simulink model "Range_ext_TCST_NoSDKF"  (R2024b)
settings: Solver=ode1  StartTime=0.0  StopTime=110000  FixedStep=5  RelTol=1e-3  EnableMultiTasking=on
values from neighbouring files (symbols this model uses):
  delta = 5    [Range_Max_2.m]    (also in Sim_Run.m; Sim_Run_Auto.m; Sim_Run_Auto_Static_SOC.m; Sim_Run_conflict_copy_danishs-macbook-air_2025_03_05.m)
  Stop_SOC = 0.1    [Sim_Run.m]    (also in Sim_Run_Auto.m; Sim_Run_Auto_Static_SOC.m; Sim_Run_conflict_copy_danishs-macbook-air_2025_03_05.m; comparison_test_weights.m)
  weights = [0.0;0.35;0.96;w_PL]    [Sim_Run.m]    (also in Sim_Run_Auto.m = [w1; w2; w3; w_PL]; Sim_Run_Auto_Static_SOC.m = [w1; w2; w3; w_PL]; Sim_Run_conflict_copy_danishs-macbook-air_2025_03_05.m = [1.0;0;0;w_PL]; comparison_test_weights.m = [w1; w2; w3; w_PL])
  x_0 = [H;M;L]    [Sim_Run.m]    (also in Sim_Run_Auto.m = [H; M; L]; Sim_Run_Auto_Static_SOC.m = [H; M; L]; Sim_Run_conflict_copy_danishs-macbook-air_2025_03_05.m; comparison_test_weights.m = [H; M; L])
settings Model: Creator=jgillis  LastModifiedBy=danish
settings SolverCC: ZeroCrossControl=DisableAll  AlgebraicLoopSolver=TrustRegion
settings DataIOCC: SaveFormat=Array  ReturnWorkspaceOutputs=off
settings OptimizationCC: LifeSpan=inf
settings DebuggingCC: UnconnectedInputMsg=warning  UnconnectedOutputMsg=warning  UnconnectedLineMsg=warning  SFUnexpectedBacktrackingDiag=warning  SFNoUnconditionalDefaultTransitionDiag=warning  ArithmeticOperatorsInVariantConditions=warning
settings HardwareCC: ProdBitPerPointer=32  ProdBitPerSizeT=32  ProdBitPerPtrDiffT=32  ProdLargestAtomicFloat=None  ProdIntDivRoundTo=Undefined  ProdEndianess=Unspecified  ProdWordSize=32  ProdHWDeviceType=32-bit Generic
settings ModelReferenceCC: EnableRefExpFcnMdlSchedulingChecks=on  PropagateSignalLabelsOutOfModel=off
settings SFSimCC: SimUseLocalCustomCode=off  CustomCodeUndefinedFunction=UseInterfaceOnly
settings RTWCC: RTWUseLocalCustomCode=off  GPUComputeCapability=3.5
settings CodeAppCC: StateflowObjectComments=on
settings GRTTargetCC: TargetLangStandard=C89/C90 (ANSI)
settings ConfigComp: CovMetricSettings=dw  CovSaveCumulativeToWorkspaceVar=on  CovSaveSingleToWorkspaceVar=on  CovExternalEMLEnable=off  CovSFcnEnable=off

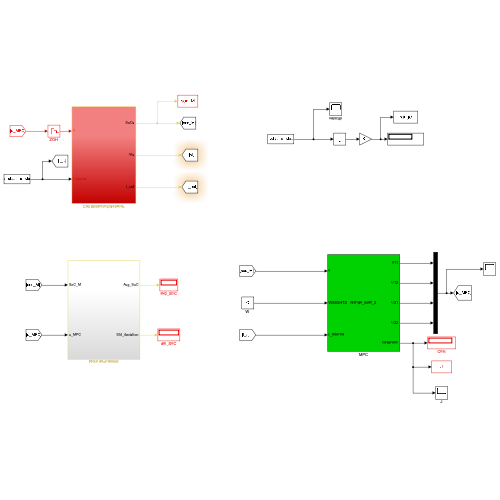
[thumbnail: Simulink's stored preview of the top-level diagram]
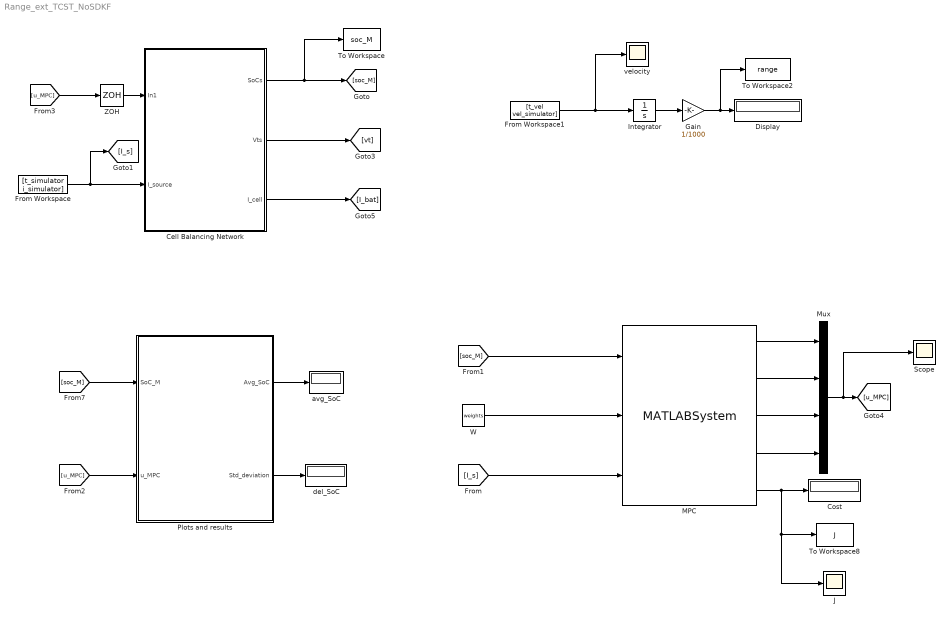
== system Range_ext_TCST_NoSDKF ==
  Cell Balancing Network : Subsystem
  Cost : Display
  Display : Display
  From Workspace : FromWorkspace  VariableName=[t_simulator i_simulator]  SampleTime=-1
  From Workspace1 : FromWorkspace  VariableName=[t_vel vel_simulator]  SampleTime=-1
  Gain : Gain  Gain=1/1000
  Integrator : Integrator
  J : Scope
  MPC : MATLABSystem  System=Range_Max_2  SimulateUsing=Interpreted execution
      mask Type: Range_Max_2
      mask Display:
      | disp('Range_Max_2');
      | port_label('input',1,'x');
      | port_label('input',2,'WEIGHTS');
      | port_label('input',3,'I_source');
      | port_label('output',1,'u11');
      | port_label('output',2,'u12');
      | port_label('output',3,'u21');
      | port_label('output',4,'u22');
      | port_label('output',5,'costFunc');
  Mux : Mux
  Plots and results : Subsystem
  Scope : Scope
  To Workspace : ToWorkspace  VariableName=soc_M  SampleTime=-1
      settings: Save2DSignal=2-D array (concatenate along first dimension)
  To Workspace2 : ToWorkspace  VariableName=range  SampleTime=-1
      settings: Save2DSignal=2-D array (concatenate along first dimension)
  To Workspace8 : ToWorkspace  VariableName=J  SampleTime=-1
      settings: Save2DSignal=2-D array (concatenate along first dimension)
  W : Constant  Value=weights
  ZOH : ZeroOrderHold  SampleTime=delta
  avg_SoC : Display
  del_SoC : Display
  velocity : Scope
  wires:
  Cell Balancing Network/2(Vts) -> [vt]
  Cell Balancing Network/1(SoCs) -> To Workspace/1, [soc_M]
  Cell Balancing Network/3(I_cell) -> [I_bat]
  [soc_M] -> MPC/1
  MPC/4 -> Mux/4
  MPC/3 -> Mux/3
  MPC/2 -> Mux/2
  MPC/1 -> Mux/1
  Mux/1 -> Scope/1, [u_MPC]
  MPC/5 -> To Workspace8/1, J/1, Cost/1
  [soc_M] -> Plots and results/1(SoC_M)
  Plots and results/1(Avg_SoC) -> avg_SoC/1
  Plots and results/2(Std_deviation) -> del_SoC/1
  ZOH/1 -> Cell Balancing Network/1(In1)
  [u_MPC] -> Plots and results/2(u_MPC)
  From Workspace1/1 -> velocity/1, Integrator/1
  Integrator/1 -> Gain/1
  Gain/1 -> To Workspace2/1, Display/1
  From Workspace/1 -> [I_s], Cell Balancing Network/2(I_source)
  [u_MPC] -> ZOH/1
  [I_s] -> MPC/3
  W/1 -> MPC/2

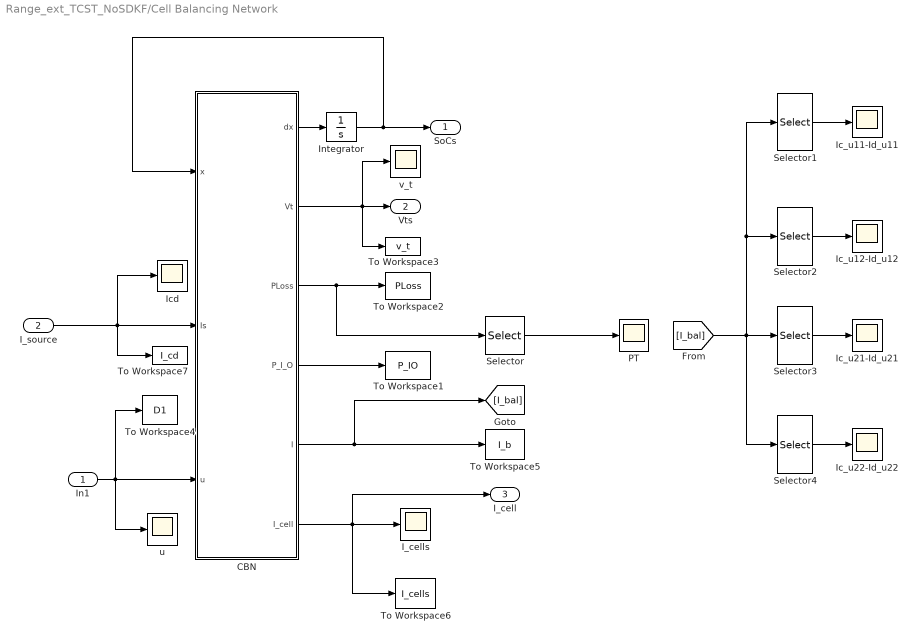
== system Range_ext_TCST_NoSDKF/Cell Balancing Network ==
  In1 : Inport
  I_source : Inport  Port=2
  CBN : MATLAB Function  TreatAsAtomicUnit=on
  I_cells : Scope
  Ic_u11-Id_u11 : Scope
  Ic_u12-Id_u12 : Scope
  Ic_u21-Id_u21 : Scope
  Ic_u22-Id_u22 : Scope
  Icd : Scope
  Integrator : Integrator  InitialCondition=x_0
  PT : Scope
  Selector : Selector  InputPortWidth=5  IndexOptions=Index vector (dialog)  Indices=1  OutputSizes=1
  Selector1 : Selector  InputPortWidth=8  IndexOptions=Index vector (dialog)  Indices=[1 2]  OutputSizes=1
  Selector2 : Selector  InputPortWidth=8  IndexOptions=Index vector (dialog)  Indices=[3 4]  OutputSizes=1
  Selector3 : Selector  InputPortWidth=8  IndexOptions=Index vector (dialog)  Indices=[5 6]  OutputSizes=1
  Selector4 : Selector  InputPortWidth=8  IndexOptions=Index vector (dialog)  Indices=[7 8]  OutputSizes=1
  To Workspace1 : ToWorkspace  VariableName=P_IO  SampleTime=-1
      settings: Save2DSignal=2-D array (concatenate along first dimension)
  To Workspace2 : ToWorkspace  VariableName=PLoss  SampleTime=-1
      settings: Save2DSignal=2-D array (concatenate along first dimension)
  To Workspace3 : ToWorkspace  VariableName=v_t  SampleTime=-1
      settings: Save2DSignal=2-D array (concatenate along first dimension)
  To Workspace4 : ToWorkspace  VariableName=D1  SampleTime=-1
      settings: Save2DSignal=2-D array (concatenate along first dimension)
  To Workspace5 : ToWorkspace  VariableName=I_b  SampleTime=-1
      settings: Save2DSignal=2-D array (concatenate along first dimension)
  To Workspace6 : ToWorkspace  VariableName=I_cells  SampleTime=-1
      settings: Save2DSignal=2-D array (concatenate along first dimension)
  To Workspace7 : ToWorkspace  VariableName=I_cd  SampleTime=-1
      settings: Save2DSignal=2-D array (concatenate along first dimension)
  u : Scope
  v_t : Scope
  SoCs : Outport
  Vts : Outport  Port=2
  I_cell : Outport  Port=3
  wires:
  CBN/1(dx) -> Integrator/1
  CBN/2(Vt) -> To Workspace3/1, Vts/1, v_t/1
  Integrator/1 -> CBN/1(x), SoCs/1
  CBN/3(PLoss) -> Selector/1, To Workspace2/1
  CBN/5(I) -> [I_bal], To Workspace5/1
  CBN/4(P_I_O) -> To Workspace1/1
  In1/1 -> To Workspace4/1, u/1, CBN/3(u)
  Selector/1 -> PT/1
  [I_bal] -> Selector4/1, Selector3/1, Selector2/1, Selector1/1
  Selector1/1 -> Ic_u11-Id_u11/1
  Selector2/1 -> Ic_u12-Id_u12/1
  CBN/6(I_cell) -> I_cell/1, To Workspace6/1, I_cells/1
  Selector3/1 -> Ic_u21-Id_u21/1
  Selector4/1 -> Ic_u22-Id_u22/1
  I_source/1 -> To Workspace7/1, Icd/1, CBN/2(Is)

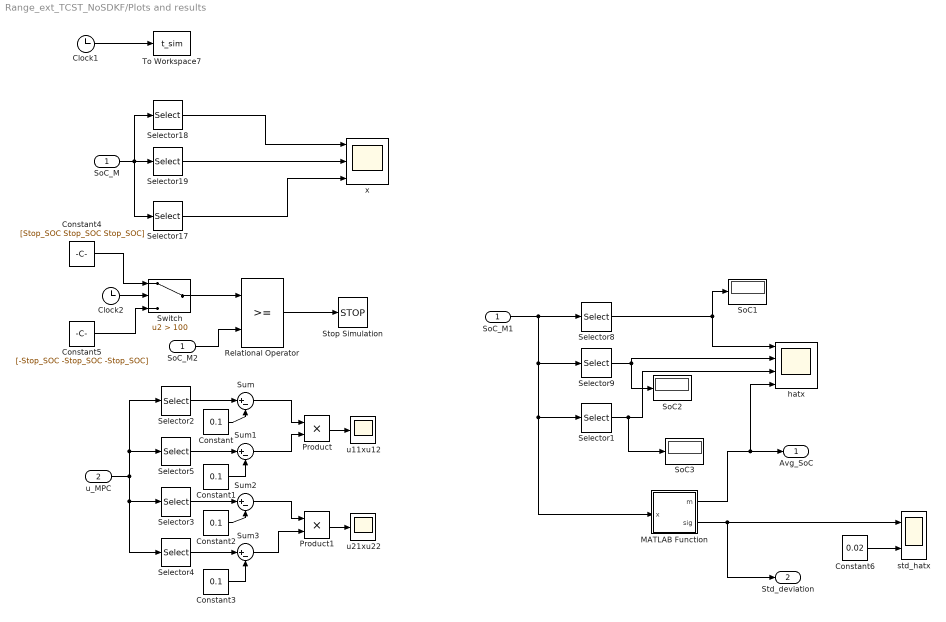
== system Range_ext_TCST_NoSDKF/Plots and results ==
  SoC_M : Inport
  u_MPC : Inport  Port=2
  Clock1 : Clock
  Clock2 : Clock
  Constant{,1..3} (4 alike) : Constant  Value=0.1
  Constant4 : Constant  Value=[Stop_SOC Stop_SOC Stop_SOC]
  Constant5 : Constant  Value=[-Stop_SOC -Stop_SOC -Stop_SOC]
  Constant6 : Constant  Value=0.02
  MATLAB Function : MATLAB Function  TreatAsAtomicUnit=on
  Product : Product
  Product1 : Product
  Relational Operator : RelationalOperator  OutDataTypeStr=boolean  InputSameDT=off
  Selector1 : Selector  InputPortWidth=3  IndexOptions=Index vector (dialog)  Indices=3  OutputSizes=1
  Selector17 : Selector  InputPortWidth=3  IndexOptions=Index vector (dialog)  Indices=3  OutputSizes=1
  Selector18 : Selector  InputPortWidth=3  IndexOptions=Index vector (dialog)  Indices=1  OutputSizes=1
  Selector19 : Selector  InputPortWidth=3  IndexOptions=Index vector (dialog)  Indices=2  OutputSizes=1
  Selector2 : Selector  InputPortWidth=4  IndexOptions=Index vector (dialog)  Indices=1  OutputSizes=1
  Selector3 : Selector  InputPortWidth=4  IndexOptions=Index vector (dialog)  Indices=3  OutputSizes=1
  Selector4 : Selector  InputPortWidth=4  IndexOptions=Index vector (dialog)  Indices=4  OutputSizes=1
  Selector5 : Selector  InputPortWidth=4  IndexOptions=Index vector (dialog)  Indices=2  OutputSizes=1
  Selector8 : Selector  InputPortWidth=3  IndexOptions=Index vector (dialog)  Indices=1  OutputSizes=1
  Selector9 : Selector  InputPortWidth=3  IndexOptions=Index vector (dialog)  Indices=2  OutputSizes=1
  SoC1 : Display
  SoC2 : Display
  SoC3 : Display
  SoC_M1 : InportShadow
  SoC_M2 : InportShadow
  Stop Simulation : Stop
  Sum{,1..3} (4 alike) : Sum  Inputs=|+-
  Switch : Switch  Criteria=u2 > Threshold  Threshold=100  SaturateOnIntegerOverflow=off  InputSameDT=off
  To Workspace7 : ToWorkspace  VariableName=t_sim  SampleTime=-1
      settings: Save2DSignal=2-D array (concatenate along first dimension)
  hatx : Scope  NumInputPorts=4
  std_hatx : Scope  NumInputPorts=2
  u11xu12 : Scope
  u21xu22 : Scope
  x : Scope  NumInputPorts=3
  Avg_SoC : Outport
  Std_deviation : Outport  Port=2
  wires:
  Selector8/1 -> SoC1/1, hatx/1
  Selector9/1 -> hatx/2, SoC2/1
  Selector1/1 -> SoC3/1, hatx/3
  MATLAB Function/2(sig) -> std_hatx/1, Std_deviation/1
  MATLAB Function/1(m) -> hatx/4, Avg_SoC/1
  u_MPC/1 -> Selector4/1, Selector3/1, Selector5/1, Selector2/1
  Product/1 -> u11xu12/1
  Product1/1 -> u21xu22/1
  Sum/1 -> Product/1
  Selector2/1 -> Sum/1
  Selector5/1 -> Sum1/1
  Sum1/1 -> Product/2
  Selector3/1 -> Sum2/1
  Selector4/1 -> Sum3/1
  Sum3/1 -> Product1/2
  Sum2/1 -> Product1/1
  Constant/1 -> Sum/2
  Constant1/1 -> Sum1/2
  Constant2/1 -> Sum2/2
  Constant3/1 -> Sum3/2
  Selector19/1 -> x/2
  SoC_M/1 -> Selector19/1, Selector18/1, Selector17/1
  Selector17/1 -> x/3
  Selector18/1 -> x/1
  Clock1/1 -> To Workspace7/1
  Relational Operator/1 -> Stop Simulation/1
  SoC_M2/1 -> Relational Operator/2
  Constant4/1 -> Switch/1
  Clock2/1 -> Switch/2
  Switch/1 -> Relational Operator/1
  Constant5/1 -> Switch/3
  Constant6/1 -> std_hatx/2
  SoC_M1/1 -> Selector1/1, MATLAB Function/1(x), Selector9/1, Selector8/1

== matlab function Range_ext_TCST_NoSDKF/Plots and results/MATLAB Function ==
  data: m output; x input; sig output
function [m,sig] = fcn(x)
%#codegen

x1=x(1);
x2=x(2);
x3=x(3);

m=(1/3)*(x1+x2+x3);
sig=sqrt((1/3)*((x1-m)^2+(x2-m)^2+(x3-m)^2));

end

== matlab function Range_ext_TCST_NoSDKF/Cell Balancing Network/CBN ==
  data: x input; Is input; u input; dx output; Vt output; PLoss output; P_I_O output; I output; I_cell output
function [dx,Vt,PLoss,P_I_O,I,I_cell ]  = CBN(x,Is,u)
%#codegen
u11=u(1);
u12=u(2);
u21=u(3);
u22=u(4);
P_I_O=zeros(2,1);
dx=zeros(3,1);
Vt=zeros(3,1);
PLoss=zeros(5,1);
I=zeros(8,1);
x1=x(1);x2=x(2);x3=x(3);
%% Constant Model Parameters 
R01=25e-3;
R02=R01;
R03=R01;
L1=6e-6; %[H], inductance
L2=6e-6; %[H], inductance
Sca1=3*3600; %[As], cell capacity
Sca2=2.7*3600; %[As], cell capacity
Sca3=2.4*3600; %[As], cell capacity
%Polynomial vector for OCV vs SoC curve
p_OCV=[88.56,-320.46,472.36,-368.96,166.57,-44.01,7.18,2.95];
%%
OCV1=0;OCV2=0;OCV3=0;
for i=1:8
OCV1=p_OCV(i)*x1^(8-i)+OCV1;
OCV2=p_OCV(i)*x2^(8-i)+OCV2;
OCV3=p_OCV(i)*x3^(8-i)+OCV3;
end
% From cell-1 to cell-2
Ic_u11=charging_current(u11,OCV1,R01,L1); % cell-1 to L1
Id_u11= discharging_current(u11,OCV1,OCV2,[R01;R02],L1);% L1 to cell-2 


% From cell-2 to cell-1
Ic_u12=charging_current(u12,OCV2,R02,L1); % cell-2 to L1 
Id_u12=discharging_current(u12,OCV2,OCV1,[R01;R02],L1); % L1 to cell-1 

%From cell-2 to cell-3
Ic_u21=charging_current(u21,OCV2,R02,L2); % cell-2 to L2
Id_u21= discharging_current(u21,OCV2,OCV3,[R02;R03],L2);% L2 to cell-3 

%From cell-3 to cell-2
Ic_u22=charging_current(u22,OCV3,R03,L2); % cell-3 to L2
Id_u22= discharging_current(u22,OCV3,OCV2,[R02;R03],L2);% L2 to cell-2 

% model dynamics
I_b1=Ic_u11+Id_u12+Is;
I_b2=Id_u11+Id_u22+Ic_u21+Ic_u12+Is;
I_b3=Ic_u22+Id_u21+Is;

dx=[(1/Sca1)*I_b1
    (1/Sca2)*I_b2
    (1/Sca3)*I_b3];
Vt=[OCV1+R01*I_b1
    OCV2+R02*I_b2
    OCV3+R03*I_b3];
I_cell=[I_b1;I_b2;I_b3];

%% power losses
%[P_cond_1,P_sw_1,P_td_1,P_R_1]=power_losses(u,H_OCV,L_OCV)
[P_cond_u11,P_sw_u11,P_td_u11,P_R_u11]=power_losses(u11,OCV1,OCV2,L1);
[P_cond_u12,P_sw_u12,P_td_u12,P_R_u12]=power_losses(u12,OCV2,OCV1,L1);


[P_cond_u21,P_sw_u21,P_td_u21,P_R_u21]=power_losses(u21,OCV2,OCV3,L2);
[P_cond_u22,P_sw_u22,P_td_u22,P_R_u22]=power_losses(u22,OCV3,OCV2,L2);


P_cond=P_cond_u11+P_cond_u12+P_cond_u21+P_cond_u22+...
       I_b1^2*R01+I_b2^2*R02+I_b3^2*R03;
P_sw=P_sw_u11+P_sw_u12+P_sw_u21+P_sw_u22;
P_td=P_td_u11+P_td_u12+P_td_u21+P_td_u22;
P_R=P_R_u11+P_R_u12+P_R_u21+P_R_u22;

PT=P_cond+P_sw+P_td+P_R;

Pin=abs(Ic_u11*OCV1+Ic_u12*OCV2+Ic_u21*OCV2+Ic_u22*OCV3);
Pout=abs(Id_u11*OCV2+Id_u12*OCV1+Id_u21*OCV3+Id_u22*OCV2);

P_I_O=[Pin;Pout];

PLoss=[PT;P_cond;P_sw;P_td;P_R];

 I=[Ic_u11
    Id_u11
    Ic_u12
    Id_u12
    Ic_u21
    Id_u21
    Ic_u22
    Id_u22];
end
